simulink model "tokamak_integrated"  (R2026a)
settings: Solver=ode3  StopTime=30  FixedStep=1e-6  MaxStep=1e-5  RelTol=1e-5
model workspace (MAT data in the model file):
  load_L2 = 0.000636619772368
  load_R2 = 0.2
undefined symbols (not defined in the file): DiscIntNeverNeededParam
libraries: ee_lib x23, nesl_utility x19, fl_lib x11, gkc_lib x1
settings Model: ModifiedByFormat=GKC3-Simulink contributors  Creator=GKC3-Simulink contributors  LastModifiedBy=GKC3-Simulink contributors

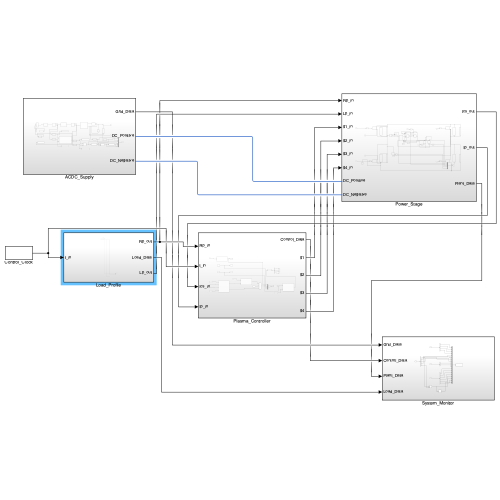
[thumbnail: Simulink's stored preview of the top-level diagram]
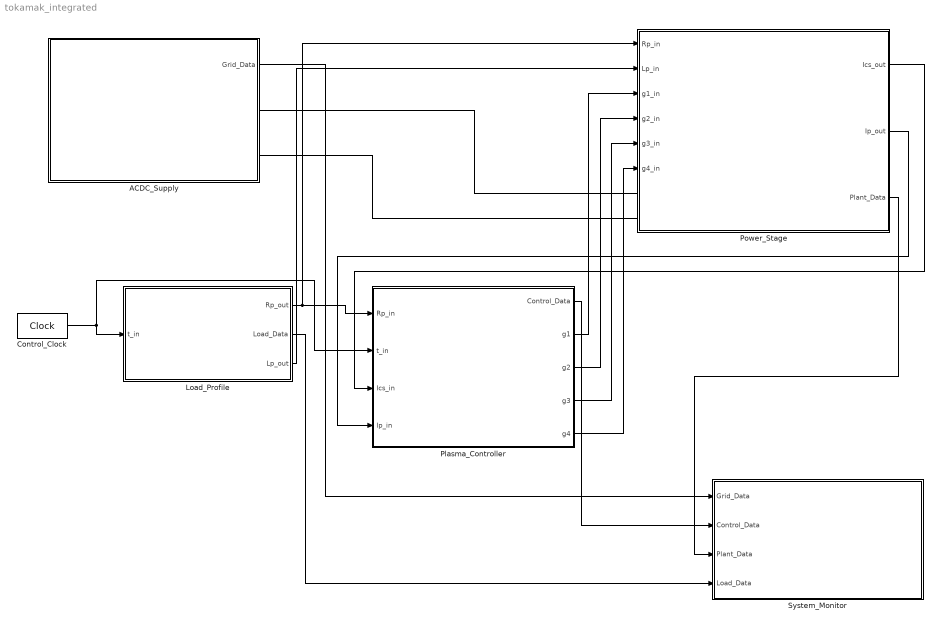
== system tokamak_integrated ==
  ACDC_Supply : Subsystem
  Control_Clock : DigitalClock  SampleTime=1e-5
  Load_Profile : Subsystem
  Plasma_Controller : Subsystem
  Power_Stage : Subsystem
  System_Monitor : Subsystem
  wires:
  Control_Clock/1 -> Load_Profile/1(t_in), Plasma_Controller/2(t_in)
  ACDC_Supply/1(Grid_Data) -> System_Monitor/1(Grid_Data)
  Plasma_Controller/1(Control_Data) -> System_Monitor/2(Control_Data)
  Plasma_Controller/2(g1) -> Power_Stage/3(g1_in)
  Plasma_Controller/3(g2) -> Power_Stage/4(g2_in)
  Plasma_Controller/4(g3) -> Power_Stage/5(g3_in)
  Plasma_Controller/5(g4) -> Power_Stage/6(g4_in)
  Power_Stage/1(Ics_out) -> Plasma_Controller/3(Ics_in)
  Power_Stage/2(Ip_out) -> Plasma_Controller/4(Ip_in)
  Power_Stage/3(Plant_Data) -> System_Monitor/3(Plant_Data)
  Load_Profile/1(Rp_out) -> Plasma_Controller/1(Rp_in), Power_Stage/1(Rp_in)
  Load_Profile/2(Load_Data) -> System_Monitor/4(Load_Data)
  Load_Profile/3(Lp_out) -> Power_Stage/2(Lp_in)
  connections:
  ACDC_Supply/RConn1 -- Power_Stage/LConn1
  ACDC_Supply/RConn2 -- Power_Stage/LConn2

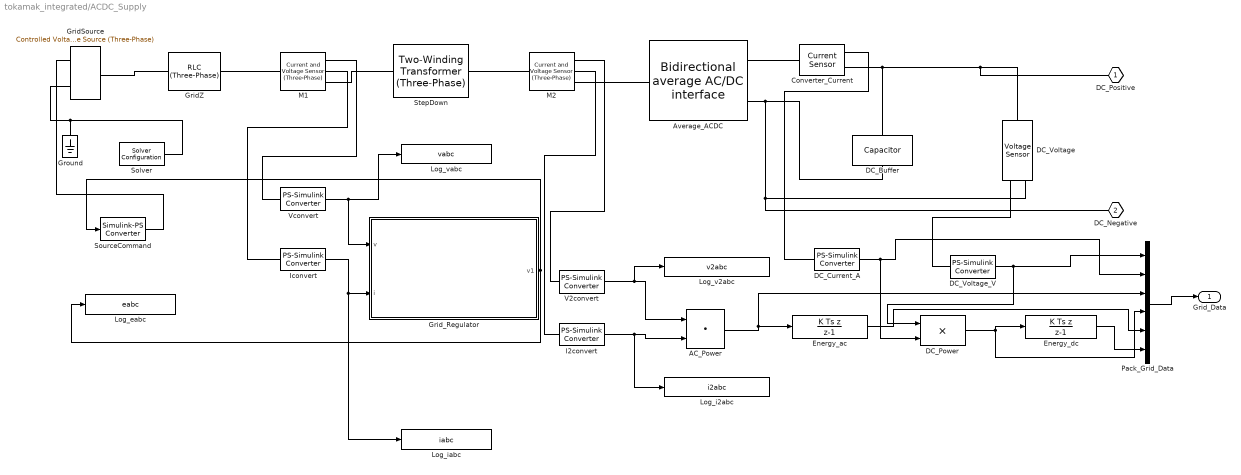
== system tokamak_integrated/ACDC_Supply ==
  AC_Power : DotProduct  OutDataTypeStr=Inherit: Inherit via internal rule
  Average_ACDC : gkc_lib/Bidirectional average AC//DC interface  voltage_ratio=2.2  frequency=50 Hz  phase=0 rad
  Converter_Current : fl_lib/Electrical/Electrical Sensors/Current Sensor
  DC_Buffer : ee_lib/Passive/Capacitor  cap_option=ee.enum.passive.capacitor.capOption.const  c=0.02 F  Cvec=[1e-05, 1e-06] F  Vvec=[0, 10] V  CV_table_symmetry=ee.enum.passive.capacitor.tableSymmetry.yes  f_vec=[1, 10] kHz  DFext_vec=[.8, 1.2]  enable_C_tol=ee.enum.toleranceApplication.none  averaging_period=0 s  C_tol=5  tol_distribution=ee.enum.toleranceDistribution.uniform  nSigma=4  r=0 Ohm  g=0 1/Ohm  enable_operating_limits=ee.enum.enable.no  operating_limit_action=ee.enum.passive.reportOpLim.warn  max_working_voltage_range=[-25, 25] V  power_rating=1 W  maxTemperature=85 degC  thermalEnable=false  thermalMass=1 J/K  i_specify=off  i_priority=None  i=0 A  i_nominal_specify=off  i_nominal_value=1  i_nominal_unit=A  v_specify=off  v_priority=None  v=0 V  v_nominal_specify=off  v_nominal_value=1  v_nominal_unit=V  vc_specify=on  vc_priority=High  vc=2200 V  vc_nominal_specify=off  vc_nominal_value=1  vc_nominal_unit=V  T_specify=off  T_priority=None  T=298.15 K  T_nominal_specify=off  T_nominal_value=1  T_nominal_unit=K
  DC_Current_A : nesl_utility/PS-Simulink Converter  PhysicalDomain=network_engine_domain  SubClassName=ps_output  LeftPortType=input  RightPortType=output  PseudoPeriodic=off  Frequencies=[]  VectorFormat=inherit  Unit=A  AffineConversion=off
  DC_Power : Product
  DC_Voltage : fl_lib/Electrical/Electrical Sensors/Voltage Sensor
  DC_Voltage_V : nesl_utility/PS-Simulink Converter  PhysicalDomain=network_engine_domain  SubClassName=ps_output  LeftPortType=input  RightPortType=output  PseudoPeriodic=off  Frequencies=[]  VectorFormat=inherit  Unit=V  AffineConversion=off
  Energy_ac : DiscreteIntegrator  IntegratorMethod=Integration: Backward Euler  SampleTime=1e-6  ICPrevOutput=DiscIntNeverNeededParam  ICPrevScaledInput=DiscIntNeverNeededParam
  Energy_dc : DiscreteIntegrator  IntegratorMethod=Integration: Backward Euler  SampleTime=1e-6  ICPrevOutput=DiscIntNeverNeededParam  ICPrevScaledInput=DiscIntNeverNeededParam
  GridSource : ee_lib/Sources/Controlled Voltage Source (Three-Phase)  Description=Implemented from the task-2 10 kV droop source guide.  input_option=ee.enum.inputType.instantaneous  FRated=50 Hz
  GridZ : ee_lib/Passive/RLC Assemblies/RLC (Three-Phase)  Description=Implemented from the task-2 10 kV droop source guide.  port_option=ee.enum.threePhasePort.composite  component_structure=ee.enum.rlc.structure.SeriesRL  R=0.1961161351 Ohm  L=0.0031212852 H  C=1e-6 F  R_parasitic=0 Ohm  G_parasitic=0 1/Ohm  IL_specify=off  IL_priority=High  IL=[0, 0, 0] A  IL_nominal_specify=off  IL_nominal_value=1  IL_nominal_unit=A  VC_specify=off  VC_priority=High  VC=[0, 0, 0] V  VC_nominal_specify=off  VC_nominal_value=1  VC_nominal_unit=V
  Grid_Regulator : Subsystem
  Ground : fl_lib/Electrical/Electrical Elements/Electrical Reference  Description=Implemented from the task-2 10 kV droop source guide.
  I2convert : nesl_utility/PS-Simulink Converter  Description=Implemented from the task-2 10 kV droop source guide.  PhysicalDomain=network_engine_domain  SubClassName=ps_output  LeftPortType=input  RightPortType=output  PseudoPeriodic=off  Frequencies=[]  VectorFormat=inherit  Unit=A  AffineConversion=off
  Iconvert : nesl_utility/PS-Simulink Converter  Description=Implemented from the task-2 10 kV droop source guide.  PhysicalDomain=network_engine_domain  SubClassName=ps_output  LeftPortType=input  RightPortType=output  PseudoPeriodic=off  Frequencies=[]  VectorFormat=inherit  Unit=A  AffineConversion=off
  Log_eabc : ToWorkspace  VariableName=eabc  SaveFormat=Timeseries  SampleTime=1e-4
      settings: Description=Implemented from the task-2 10 kV droop source guide.
  Log_i2abc : ToWorkspace  VariableName=i2abc  SaveFormat=Timeseries  SampleTime=1e-4
      settings: Description=Implemented from the task-2 10 kV droop source guide.
  Log_iabc : ToWorkspace  VariableName=iabc  SaveFormat=Timeseries  SampleTime=1e-4
      settings: Description=Implemented from the task-2 10 kV droop source guide.
  Log_v2abc : ToWorkspace  VariableName=v2abc  SaveFormat=Timeseries  SampleTime=1e-4
      settings: Description=Implemented from the task-2 10 kV droop source guide.
  Log_vabc : ToWorkspace  VariableName=vabc  SaveFormat=Timeseries  SampleTime=1e-4
      settings: Description=Implemented from the task-2 10 kV droop source guide.
  M1 : ee_lib/Sensors & Transducers/Current and Voltage Sensor (Three-Phase)  Description=10 kV bus measurement downstream of grid impedance; current positive toward load.  port_option=ee.enum.threePhasePort.composite  vMeasurementType=ee.enum.vmeasurement.lg  outputUnit=ee.enum.unit.si  SRated=100e6 A*V  VRated=24e3 V  I_specify=off  I_priority=None  I=[0, 0, 0] A  I_nominal_specify=off  I_nominal_value=1  I_nominal_unit=A  V_specify=off  V_priority=None  V=[0, 0, 0] V  V_nominal_specify=off  V_nominal_value=1  V_nominal_unit=V
  M2 : ee_lib/Sensors & Transducers/Current and Voltage Sensor (Three-Phase)  Description=Implemented from the task-2 10 kV droop source guide.  port_option=ee.enum.threePhasePort.composite  vMeasurementType=ee.enum.vmeasurement.lg  outputUnit=ee.enum.unit.si  SRated=100e6 A*V  VRated=24e3 V  I_specify=off  I_priority=None  I=[0, 0, 0] A  I_nominal_specify=off  I_nominal_value=1  I_nominal_unit=A  V_specify=off  V_priority=None  V=[0, 0, 0] V  V_nominal_specify=off  V_nominal_value=1  V_nominal_unit=V
  Pack_Grid_Data : Mux  Inputs=6
  Solver : nesl_utility/Solver Configuration  Description=Implemented from the task-2 10 kV droop source guide.  PhysicalDomain=network_engine_domain  SubClassName=solver  LeftPortType=input  RightPortType=generic  Tones=[]  Harmonics=[]  SimulateNoise=off  Profile=off  UseLocalSampling=off  EnableSwitchedLinearOptims=on  FrequencyDomain=off  UseCCode=off  RelTol=0.001  AbsTol=0.001  MinStep=1e-09  ToWorkspace=off  RevertToSquareIcSolve=off  NumHomotopyIterations=100  PhasorMode=off  PhasorModeNumHarmonics=1  ConsistencySolver=NEWTON_XTOL_AFTER_FTOL  CanonicalOrdering=CANONICAL  OptimizeIntermediates=OPTIMIZED  IndexReductionMethod=DerivativeReplacement  DoDC=off  ResidualTolerance=1e-09  ConsistencyTolSource=GLOBAL  ConsistencyAbsTol=0.001  ConsistencyRelTol=0.001  ConsistencyTolFactor=0.001  UseLocalSolver=on  LocalSolverChoice=NE_BACKWARD_EULER_ADVANCER  ResolveIndetEquations=on  FunctionEvalNumThread=1  LocalSolverSampleTime=1e-6  DoFixedCost=on  MaxNonlinIter=3  MaxModeIter=2  ComputeImpulses=off  ImpulseIterations=2  LinearAlgebra=Sparse  LinearAlgebraNumThread=0  EquationFormulation=NE_TIME_EF  DelaysMemoryBudget=1024  AutomaticFiltering=on  FilteringTimeConstant=0.001  PartitionStorageMethod=AS_NEEDED  PartitionMemoryBudget=1024  PartitionMethod=ROBUST  MultibodyUseLocalSolver=off  MultibodyLocalSolverChoice=ODE1  MultibodyLocalSolverSampleTime=0.001
  SourceCommand : nesl_utility/Simulink-PS Converter  Description=Implemented from the task-2 10 kV droop source guide.  PhysicalDomain=network_engine_domain  SubClassName=ps_input  LeftPortType=input  RightPortType=output  PseudoPeriodic=off  Frequencies=[]  NoiseDistribution=none  NoiseParameters=[]  Unit=V  AffineConversion=off  FilteringAndDerivatives=provide  SimscapeFilterOrder=1  InputFilterTimeConstant=0.001  UdotUserProvided=0
  StepDown : ee_lib/Passive/Transformers/Two-Winding Transformer (Three-Phase)  Description=Validation transformer: 10 kV/1000 V, 10 MVA, Yg/Yg, winding R 1e-6 pu each; no leakage/magnetization/saturation.  SRated=10e6 A*V  FRated=50 Hz  Winding1Connection=ee.enum.windingconnection.Yg  VRated1=10000 V  Winding2Connection=ee.enum.windingconnection.Yg  VRated2=1000 V  CoreType=ee.enum.coretype.threelimb  pu_Rw1=1e-6  pu_Rw2=1e-6  leakage_reactance_option=ee.enum.transformer_leakage.exclude  pu_Xl1=0.05  pu_Xl2=0.05  magnetizing_resistance_option=ee.enum.transformer_magnetizingResistance.exclude  pu_Rm=500  magnetizing_reactance_option=ee.enum.transformer_magnetizingReactance.exclude  saturation_option=ee.enum.transformer_saturation.exclude  pu_Xm=500  current_data=[0, .002, 1, 2]  magnetic_flux_data=[0, 1.2, 1.5, 1.51]  pu_X0=0.5  i1_specify=off  i1_priority=None  i1=[0, 0, 0] A  i1_nominal_specify=off  i1_nominal_value=1  i1_nominal_unit=A  i2_specify=off  i2_priority=None  i2=[0, 0, 0] A  i2_nominal_specify=off  i2_nominal_value=1  i2_nominal_unit=A  phi_specify=off  phi_priority=None  phi=[0, 0, 0]  phi_nominal_specify=off  phi_nominal_value=1  phi_nominal_unit=1
  V2convert : nesl_utility/PS-Simulink Converter  Description=Implemented from the task-2 10 kV droop source guide.  PhysicalDomain=network_engine_domain  SubClassName=ps_output  LeftPortType=input  RightPortType=output  PseudoPeriodic=off  Frequencies=[]  VectorFormat=inherit  Unit=V  AffineConversion=off
  Vconvert : nesl_utility/PS-Simulink Converter  Description=Implemented from the task-2 10 kV droop source guide.  PhysicalDomain=network_engine_domain  SubClassName=ps_output  LeftPortType=input  RightPortType=output  PseudoPeriodic=off  Frequencies=[]  VectorFormat=inherit  Unit=V  AffineConversion=off
  DC_Positive : PMIOPort  Side=Right
  DC_Negative : PMIOPort  Port=2  Side=Right
  Grid_Data : Outport
  wires:
  DC_Power/1 -> Pack_Grid_Data/4, Energy_dc/1
  Energy_dc/1 -> Pack_Grid_Data/6
  Pack_Grid_Data/1 -> Grid_Data/1
  DC_Current_A/1 -> Pack_Grid_Data/2, DC_Power/2
  AC_Power/1 -> Pack_Grid_Data/3, Energy_ac/1
  DC_Voltage_V/1 -> Pack_Grid_Data/1, DC_Power/1
  Energy_ac/1 -> Pack_Grid_Data/5
  Grid_Regulator/1(v1) -> SourceCommand/1, Log_eabc/1
  V2convert/1 -> Log_v2abc/1, AC_Power/1
  I2convert/1 -> Log_i2abc/1, AC_Power/2
  Iconvert/1 -> Log_iabc/1, Grid_Regulator/2(i)
  Vconvert/1 -> Log_vabc/1, Grid_Regulator/1(v)
  connections:
  DC_Voltage/RConn2 -- Average_ACDC/RConn2 -- DC_Buffer/RConn1 -- DC_Negative/RConn1
  Converter_Current/RConn2 -- DC_Positive/RConn1 -- DC_Voltage/LConn1 -- DC_Buffer/LConn1
  Solver/RConn1 -- Ground/LConn1 -- GridSource/LConn2
  M2/RConn2 -- I2convert/LConn1
  M1/RConn1 -- Vconvert/LConn1
  GridZ/RConn1 -- M1/LConn1
  M1/RConn3 -- StepDown/LConn1
  GridSource/RConn1 -- GridZ/LConn1
  StepDown/RConn1 -- M2/LConn1
  DC_Voltage/RConn1 -- DC_Voltage_V/LConn1
  M2/RConn1 -- V2convert/LConn1
  M1/RConn2 -- Iconvert/LConn1
  SourceCommand/RConn1 -- GridSource/LConn1
  Average_ACDC/RConn1 -- Converter_Current/LConn1
  Converter_Current/RConn1 -- DC_Current_A/LConn1
  M2/RConn3 -- Average_ACDC/LConn1

== system tokamak_integrated/Load_Profile ==
  t_in : Inport
  Lp_schedule : Lookup_n-D  NumberOfTableDimensions=1  BreakpointsForDimension1=[0 0.6 1.6 30]  Table=[150e-6 150e-6 100e-6 100e-6]  ExtrapMethod=Clip  InternalRulePriority=Speed  RndMeth=Simplest
  Pack_Load_Data : Mux  Inputs=2
  Rp_schedule : Lookup_n-D  NumberOfTableDimensions=1  BreakpointsForDimension1=[0 0.6 1.6 11.6 12.1 12.3 30]  Table=[0.015 0.015 0.01 0.01 0.01 100 100]  ExtrapMethod=Clip  InternalRulePriority=Speed  RndMeth=Simplest
  Rp_out : Outport
  Load_Data : Outport  Port=2
  Lp_out : Outport  Port=3
  wires:
  Rp_schedule/1 -> Pack_Load_Data/1, Rp_out/1
  Pack_Load_Data/1 -> Load_Data/1
  Lp_schedule/1 -> Lp_out/1, Pack_Load_Data/2
  t_in/1 -> Rp_schedule/1, Lp_schedule/1

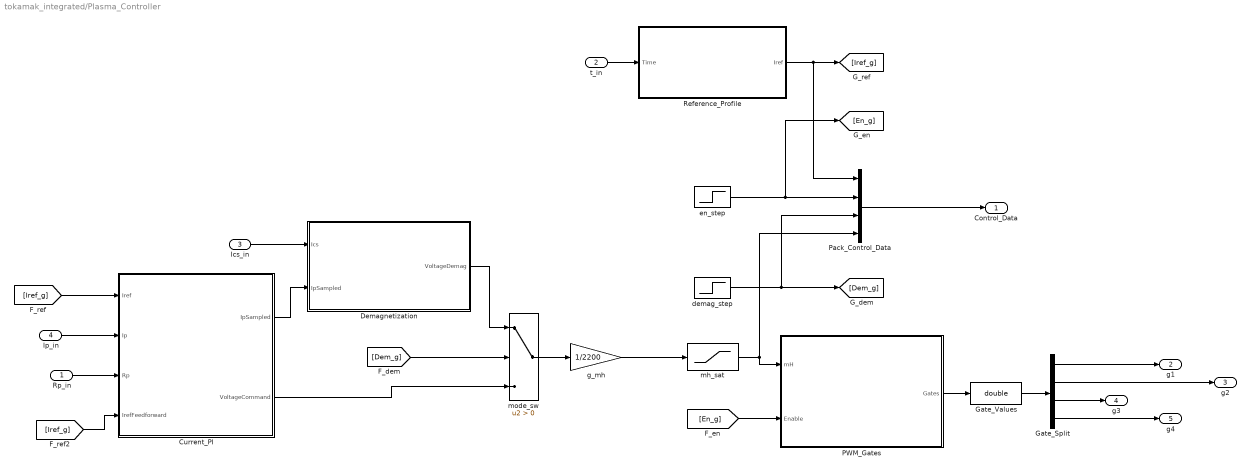
== system tokamak_integrated/Plasma_Controller ==
  Rp_in : Inport
  t_in : Inport  Port=2
  Ics_in : Inport  Port=3
  Ip_in : Inport  Port=4
  Current_PI : Subsystem
  Demagnetization : Subsystem
  Gate_Split : Demux
  Gate_Values : DataTypeConversion  OutDataTypeStr=double  SaturateOnIntegerOverflow=off  RndMeth=Floor
  PWM_Gates : Subsystem
  Pack_Control_Data : Mux
  Reference_Profile : Subsystem
  demag_step : Step  Time=12.3  SampleTime=0
  en_step : Step  Time=0.6  SampleTime=0
  g_mh : Gain  Gain=1/2200
  mh_sat : Saturate  UpperLimit=0.95  LowerLimit=-0.95
  mode_sw : Switch  Criteria=u2 > Threshold  SaturateOnIntegerOverflow=off  InputSameDT=off
  Control_Data : Outport
  g1 : Outport  Port=2
  g2 : Outport  Port=3
  g3 : Outport  Port=4
  g4 : Outport  Port=5
  wires:
  g_mh/1 -> mh_sat/1
  t_in/1 -> Reference_Profile/1(Time)
  [Iref_g] -> Current_PI/1(Iref)
  Ip_in/1 -> Current_PI/2(Ip)
  Rp_in/1 -> Current_PI/3(Rp)
  [Iref_g] -> Current_PI/4(IrefFeedforward)
  Current_PI/2(VoltageCommand) -> mode_sw/3
  Ics_in/1 -> Demagnetization/1(Ics)
  Current_PI/1(IpSampled) -> Demagnetization/2(IpSampled)
  Demagnetization/1(VoltageDemag) -> mode_sw/1
  [En_g] -> PWM_Gates/2(Enable)
  [Dem_g] -> mode_sw/2
  mode_sw/1 -> g_mh/1
  Pack_Control_Data/1 -> Control_Data/1
  Gate_Split/3 -> g3/1
  Gate_Split/1 -> g1/1
  PWM_Gates/1(Gates) -> Gate_Values/1
  Reference_Profile/1(Iref) -> [Iref_g], Pack_Control_Data/1
  mh_sat/1 -> PWM_Gates/1(mH), Pack_Control_Data/4
  Gate_Split/2 -> g2/1
  Gate_Split/4 -> g4/1
  Gate_Values/1 -> Gate_Split/1
  en_step/1 -> [En_g], Pack_Control_Data/2
  demag_step/1 -> [Dem_g], Pack_Control_Data/3

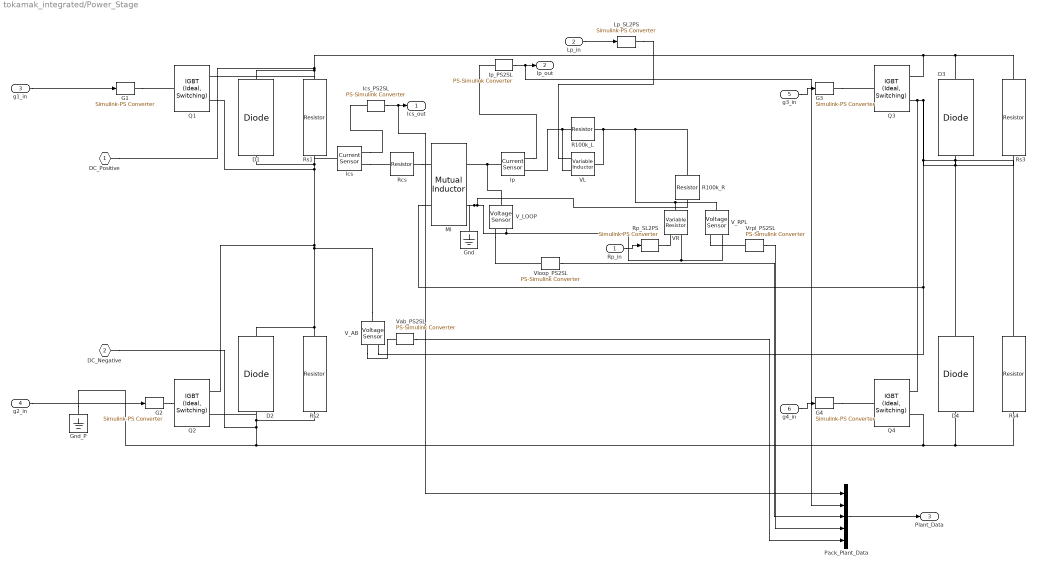
== system tokamak_integrated/Power_Stage ==
  Rp_in : Inport
  Lp_in : Inport  Port=2
  g1_in : Inport  Port=3
  g2_in : Inport  Port=4
  g3_in : Inport  Port=5
  g4_in : Inport  Port=6
  D{1..4} (4 alike) : ee_lib/Semiconductors & Converters/Diode  ModelType=ee.enum.diode.modelType.pwl  TableType=ee.enum.diode.tableType.IfMat  IfMat=[.07, .12, .19, 1.75, 4.24, 7.32, 11.2; .16, .3, .72, 2.14, 5.02, 8.35, 13.12] A  VfMat=[.9, 1.15, 1.25, 1.5, 1.75, 2.17, 2.6, 2.85; .58, .68, .75, 1.1, 1.38, 1.77, 2.27, 2.7] V  TjVec=[25, 125] degC  VfVec=[.5, .7, .9, 1.3, 1.7, 2.1, 2.5] V  IfVec=[.1, .2, .5, 1, 2, 4, 7, 10] A  IrMat=[1e-06, 2e-06, 5e-06, 1e-05, 2.5e-05, 5e-05, .0001; 2e-06, 5e-06, 1e-05, 4e-05, 8e-05, .0002, .0005] A  VrMat=[10, 100, 200, 250, 300, 325, 350; 10, 70, 160, 220, 270, 300, 320] V  VrVec=[10, 20, 40, 50, 70, 80, 100] V  IrVec=[1e-06, 2e-06, 5e-06, 1e-05, 2e-05, 5e-05, .0001] A  Vf=2 V  Ron=20e-6 Ohm  Goff=1e-8 S  prmExp=ee.enum.diode.expParam.useTwo  I12=[.0137, .545] A  V12=[.6, .7] V  RS=0 Ohm  Tmeas=298.15 K  IS=1e-12 A  ec=1  I1=0.0137 A  V1=0.6 V  N_series=1  N_parallel=1  ZenerEnable=false  Rz=0.3 Ohm  BV=30 V  C_param=ee.enum.diode.capParam.fixed  CJ=0 pF  CJ0=5 pF  Vvec=[.1, 10, 100] V  Cvec=[3.5, 1, .4] pF  VJ=1 V  Mgrad=0.5  FC=0.5  Q_param=ee.enum.diode.recoveryParam.off  iRM=-7.15 A  iF=4 A  didt=-750 A/us  trr_factor=3  trr=115 ns  Qrr=150 nA*s  Vr=-600 V  Ls=150 nH  Erec=0.03 J  TT=50 ns  tau=100 ns  T_param=ee.enum.diode.temperatureParam.off  Tdevice=298.15 K  I1_T2=0.245 A  V1_T2=0.5 V  IS_T2=1.25e-7 A  Tmeas2=125 degC  XTI_param=ee.enum.diode.xtiParam.pn  XTI=3  EG_param=ee.enum.diode.egapParam.material_si  EG=1.11 eV  dBVdT=0 V/K  enable_fault_input=simscape.enum.onoff.off  i_specify=off  i_priority=None  i=0 A  i_nominal_specify=off  i_nominal_value=1  i_nominal_unit=A  v_specify=off  v_priority=None  v=0 V  v_nominal_specify=off  v_nominal_value=1  v_nominal_unit=V  v_capacitor_specify=off  v_capacitor_priority=None  v_capacitor=0 V  v_capacitor_nominal_specify=off  v_capacitor_nominal_value=1  v_capacitor_nominal_unit=V  Qj_specify=off  Qj_priority=High  Qj=0 C  Qj_nominal_specify=off  Qj_nominal_value=1  Qj_nominal_unit=C  i_diode_specify=off  i_diode_priority=None  i_diode=0 A  i_diode_nominal_specify=off  i_diode_nominal_value=1  i_diode_nominal_unit=A  v_diode_specify=off  v_diode_priority=None  v_diode=0 V  v_diode_nominal_specify=off  v_diode_nominal_value=1  v_diode_nominal_unit=V  i_capacitor_specify=off  i_capacitor_priority=None  i_capacitor=0 A  i_capacitor_nominal_specify=off  i_capacitor_nominal_value=1  i_capacitor_nominal_unit=A  fidelity_level=ee.enum.diode.fidelity.includeChargeDyn  rec_loss_model=ee.enum.diode.reverseRecoveryModelTabulateUpTo3D.fixed  ErecVal=0 J  scaleWithIandV=true  ErecMat=zeros(2, 3) J  ErecMat3D=zeros(2, 3, 2) J  TjrecVec=[298.15, 398.15] K  IfrecVec=[.1, 1, 10] A  IrecVal=10 A  VrecVal=10 V  VrecVec=[0, 100] V  tFilter=1 / 1000 / 100 s  thermal_network_parameterization=ee.enum.thermalNetworkTopology.junctionCase  Rth=[0, 10] K/W  Rth_Cauer=[1, 3, 10] K/W  Rth_Foster=[.08, .14, .22, .16] K/W  thermal_mass_parameterization=ee.enum.thermalNetwork.timeconstant  thermal_mass=[0, 1] J/K  thermal_mass_Cauer=[.1, .3, 1] J/K  thermal_mass_Foster=[.001, .005, .05, .5] J/K  thermal_time_constant=[0, 10] s  thermal_time_constant_Cauer=[1, 3, 10] s  thermal_time_constant_Foster=[7e-05, .0007, .01, .08] s  thermal_mass_initial_temperatures=[25, 25] degC  thermal_mass_initial_temperatures_Cauer=[25, 25, 25] degC  junction_thermal_mass=0.01 J/K  Tvec_initial_Foster=[25, 25, 25, 25] degC  no_thermal_network=0  junction_temperature_specify=off  junction_temperature_priority=None  junction_temperature=25 degC  junction_temperature_nominal_specify=off  junction_temperature_nominal_value=1  junction_temperature_nominal_unit=degC
  G{1..4} (4 alike) : nesl_utility/Simulink-PS Converter  PhysicalDomain=network_engine_domain  SubClassName=ps_input  LeftPortType=input  RightPortType=output  PseudoPeriodic=off  Frequencies=[]  NoiseDistribution=none  NoiseParameters=[]  Unit=V  AffineConversion=off  FilteringAndDerivatives=zero  SimscapeFilterOrder=1  InputFilterTimeConstant=0.001  UdotUserProvided=0
  Gnd : fl_lib/Electrical/Electrical Elements/Electrical Reference
  Gnd_P : fl_lib/Electrical/Electrical Elements/Electrical Reference
  Ics : fl_lib/Electrical/Electrical Sensors/Current Sensor
  Ics_PS2SL : nesl_utility/PS-Simulink Converter  PhysicalDomain=network_engine_domain  SubClassName=ps_output  LeftPortType=input  RightPortType=output  PseudoPeriodic=off  Frequencies=[]  VectorFormat=inherit  Unit=A  AffineConversion=off
  Ip : fl_lib/Electrical/Electrical Sensors/Current Sensor
  Ip_PS2SL : nesl_utility/PS-Simulink Converter  PhysicalDomain=network_engine_domain  SubClassName=ps_output  LeftPortType=input  RightPortType=output  PseudoPeriodic=off  Frequencies=[]  VectorFormat=inherit  Unit=A  AffineConversion=off
  Lp_SL2PS : nesl_utility/Simulink-PS Converter  PhysicalDomain=network_engine_domain  SubClassName=ps_input  LeftPortType=input  RightPortType=output  PseudoPeriodic=off  Frequencies=[]  NoiseDistribution=none  NoiseParameters=[]  Unit=H  AffineConversion=off  FilteringAndDerivatives=provide  SimscapeFilterOrder=1  InputFilterTimeConstant=0.001  UdotUserProvided=0
  MI : ee_lib/Passive/Transformers/Mutual Inductor  L1=1 H  L2=1 H  k=0.99999  L_tol=20  enable_L1_tol=ee.enum.toleranceApplication.none  L1_tol_distribution=ee.enum.toleranceDistribution.uniform  L1_nSigma=4  enable_L2_tol=ee.enum.toleranceApplication.none  L2_tol_distribution=ee.enum.toleranceDistribution.uniform  L2_nSigma=4  r=[1e-9, 1e-9] Ohm  g=[1e-9, 1e-9] 1/Ohm  enable_operating_limits=ee.enum.enable.no  operating_limit_action=ee.enum.passive.reportOpLim.warn  max_working_current=1 A  power_rating=1 W  iL1_specify=off  iL1_priority=High  iL1=0 A  iL1_nominal_specify=off  iL1_nominal_value=1  iL1_nominal_unit=A  iL2_specify=off  iL2_priority=High  iL2=0 A  iL2_nominal_specify=off  iL2_nominal_value=1  iL2_nominal_unit=A
  Pack_Plant_Data : Mux  Inputs=5
  Q{1..4} (4 alike) : ee_lib/Semiconductors & Converters/IGBT (Ideal, Switching)  port_option=ee.enum.controlport.ps  Vf=2 V  Ron=20e-6 Ohm  Goff=1e-8 1/Ohm  Vth=0.5 V  diode_param=ee.enum.semiconductors.protectionDiode.external  diode_Vf=0.8 V  diode_Ron=0.001 Ohm  diode_Goff=1e-5 1/Ohm  diode_C=50e-9 F  diode_iRM=-235 A  diode_iF=300 A  diode_idot=-50 A/us  diode_trr_param=ee.enum.converters.diodeReverseParam.trr_factor  diode_trr_factor=3  diode_trr=15 us  diode_Qrr=1500 s*uA  ice_specify=off  ice_priority=None  ice=0 A  ice_nominal_specify=off  ice_nominal_value=1  ice_nominal_unit=A  vce_specify=off  vce_priority=None  vce=0 V  vce_nominal_specify=off  vce_nominal_value=1  vce_nominal_unit=V  vge_specify=off  vge_priority=None  vge=0 V  vge_nominal_specify=off  vge_nominal_value=1  vge_nominal_unit=V  thermal_loss_option=ee.enum.converters.thermalLossOption.constantvalues  Von_data=[0, .1, .6, .8, 1, 1.3, 1.6, 2, 2.4; 0, .1, .7, 1, 1.2, 1.5, 1.9, 2.4, 2.8] V  Tj=[298.15, 398.15] K  Iout_data=[0, .1, 1, 5, 10, 20, 40, 70, 100] A  tabulateWithVce=false  Eon_data=[0, .0024, .024, .12, .2, .48, 1.04, 2.16, 3.24; 0, .003, .03, .15, .25, .6, 1.3, 2.7, 4.05] * 1e-3 J  Eoff_data=[0, .0007, .0066, .033, .066, .17, .33, .83, 1.5; 0, .001, .01, .05, .1, .25, .5, 1.2, 2.2] * 1e-3 J  Eon_data_3D=[zeros(2, 9, 3)] J  Eoff_data_3D=[zeros(2, 9, 3)] J  Tj_loss=[298.15, 398.15] K  Iout_data_loss=[0, .1, 1, 5, 10, 20, 40, 70, 100] A  Vce_loss=[0, 150, 300] V  Eon_scalar=22.86e-3 J  Eoff_scalar=17.14e-3 J  Voff=300 V  Iout_scalar=600 A  useCurrentFromPreviousCycle=false  useVoltageFromPreviousCycle=false  diodeModelType=ee.enum.converters.diodeModelType.pwl  diodeTableType=ee.enum.diode.tableType.IfMat  diode_ReverseIVType=ee.enum.diode.diodeReverseIV.constant  diode_IfMat=[.07, .12, .19, 1.75, 4.24, 7.32, 11.2; .16, .3, .72, 2.14, 4.02, 6.35, 9.12] A  diode_VfMat=[.9, 1.15, 1.25, 1.5, 1.75, 2.17, 2.6, 2.85; .58, .68, .75, 1.1, 1.38, 1.77, 2.27, 2.7] V  diode_TjVec=[25, 125] degC  diode_VfVec=[.5, .7, .9, 1.3, 1.7, 2.1, 2.5] V  diode_IfVec=[.1, .2, .5, 1, 2, 4, 7, 10] A  diode_IrMat=[1e-06, 2e-06, 5e-06, 1e-05, 2.5e-05, 5e-05, .0001; 2e-06, 5e-06, 1e-05, 4e-05, 8e-05, .0002, .0005] A  diode_VrMat=[10, 100, 200, 250, 300, 325, 350; 10, 70, 160, 220, 270, 300, 320] V  diode_VrVec=[10, 20, 40, 50, 70, 80, 100] V  diode_IrVec=[1e-06, 2e-06, 5e-06, 1e-05, 2e-05, 5e-05, .0001] A  diode_Vr=-600 V  diode_Ls=150 nH  diode_Erec=0.03 J  diode_rec_loss_model=ee.enum.diode.reverseRecoveryModelTabulateUpTo3D.fixed  diode_ErecVal=0 J  diode_scaleWithIandV=true  diode_ErecMat=zeros(2, 3) J  diodeErecMat3D=zeros(2, 3, 2) J  diode_TjrecVec=[298.15, 398.15] K  diode_IfrecVec=[.1, 1, 10] A  diodeVrecVec=[0, 100] V  diode_IrecVal=10 A  diode_VrecVal=10 V  diode_tFilter=1 / 1000 / 100 s  separateThermalPortForDiode=false  thermal_network_parameterization=ee.enum.thermalNetworkTopology.external  Rth=[.08, .5] K/W  Rth_Cauer=[.08, .1, .5] K/W  Rth_Foster=[.08, .14, .22, .16] K/W  thermal_mass_parameterization=ee.enum.thermalNetwork.timeconstant  thermal_mass=[.01, .5] J/K  thermal_mass_Cauer=[.01, .1, .5] J/K  thermal_mass_Foster=[.001, .005, .05, .5] J/K  thermal_time_constant=[.001, .2] s  thermal_time_constant_Cauer=[.001, .1, .2] s  thermal_time_constant_Foster=[7e-05, .0007, .01, .08] s  thermal_mass_initial_temperatures=[25, 25] degC  thermal_mass_initial_temperatures_Cauer=[25, 25, 25] degC  junction_thermal_mass=0.01 J/K  Tvec_initial_Foster=[25, 25, 25, 25] degC  RthDiode=[.03, .2] K/W  RthCauerDiode=[.03, .1, .2] K/W  RthFosterDiode=[.03, .2] K/W  thermalMassDiode=[3, 25] J/K  thermalMassCauerDiode=[3, 10, 25] J/K  thermalMassFosterDiode=[33, 50] J/K  thermalTauDiode=[.1, 5] s  thermalTauCauerDiode=[.1, 1, 5] s  thermalTauFosterDiode=[1, 10] s  thermalMassInitTempDiode=[25, 25] degC  thermalMassInitTempCauerDiode=[25, 25, 25] degC  junctionthermalMassDiode=0.1 J/K  TVecInitialFosterDiode=[25, 25, 25, 25] degC  no_thermal_network=ee.enum.enable.no  IGBT_junction_temperature_specify=off  IGBT_junction_temperature_priority=None  IGBT_junction_temperature=25 degC  IGBT_junction_temperature_nominal_specify=off  IGBT_junction_temperature_nominal_value=1  IGBT_junction_temperature_nominal_unit=degC  diode_junction_temperature_specify=off  diode_junction_temperature_priority=None  diode_junction_temperature=25 degC  diode_junction_temperature_nominal_specify=off  diode_junction_temperature_nominal_value=1  diode_junction_temperature_nominal_unit=degC  Qj_specify=off  Qj_priority=None  Qj=0 W  Qj_nominal_specify=off  Qj_nominal_value=1  Qj_nominal_unit=W  accumulatedSwitchingLosses_specify=off  accumulatedSwitchingLosses_priority=None  accumulatedSwitchingLosses=0 J
  R100k_L : ee_lib/Passive/Resistor  R=1e5 Ohm  enable_R_tol=ee.enum.toleranceApplication.none  R_tol=5  tol_distribution=ee.enum.toleranceDistribution.uniform  nSigma=4  enable_operating_limits=ee.enum.enable.no  operating_limit_action=ee.enum.passive.reportOpLim.warn  power_rating=1 W  max_working_voltage=100 V  noise_mode=ee.enum.sources.noise.Disabled  Tdevice=25 degC  sample_time=1e-3 s  repeatability=ee.enum.ic.repeatability.notRepeatable  user_seed=0  auto_seed=817904655  power_derating_T1=70 degC  power_derating_T2=155 degC  operating_temperature_range_vec=[-50, 150] degC  alpha=3.93e-3 1/K  Tmeas=25 degC  thermal_mass=100 J/K  temperature_specify=off  temperature_priority=High  temperature=298.15 K  temperature_nominal_specify=off  temperature_nominal_value=1  temperature_nominal_unit=K
  R100k_R : ee_lib/Passive/Resistor  R=1e5 Ohm  enable_R_tol=ee.enum.toleranceApplication.none  R_tol=5  tol_distribution=ee.enum.toleranceDistribution.uniform  nSigma=4  enable_operating_limits=ee.enum.enable.no  operating_limit_action=ee.enum.passive.reportOpLim.warn  power_rating=1 W  max_working_voltage=100 V  noise_mode=ee.enum.sources.noise.Disabled  Tdevice=25 degC  sample_time=1e-3 s  repeatability=ee.enum.ic.repeatability.notRepeatable  user_seed=0  auto_seed=1584484500  power_derating_T1=70 degC  power_derating_T2=155 degC  operating_temperature_range_vec=[-50, 150] degC  alpha=3.93e-3 1/K  Tmeas=25 degC  thermal_mass=100 J/K  temperature_specify=off  temperature_priority=High  temperature=298.15 K  temperature_nominal_specify=off  temperature_nominal_value=1  temperature_nominal_unit=K
  Rcs : ee_lib/Passive/Resistor  R=20e-6 Ohm  enable_R_tol=ee.enum.toleranceApplication.none  R_tol=5  tol_distribution=ee.enum.toleranceDistribution.uniform  nSigma=4  enable_operating_limits=ee.enum.enable.no  operating_limit_action=ee.enum.passive.reportOpLim.warn  power_rating=1 W  max_working_voltage=100 V  noise_mode=ee.enum.sources.noise.Disabled  Tdevice=25 degC  sample_time=1e-3 s  repeatability=ee.enum.ic.repeatability.notRepeatable  user_seed=0  auto_seed=1978802833  power_derating_T1=70 degC  power_derating_T2=155 degC  operating_temperature_range_vec=[-50, 150] degC  alpha=3.93e-3 1/K  Tmeas=25 degC  thermal_mass=100 J/K  temperature_specify=off  temperature_priority=High  temperature=298.15 K  temperature_nominal_specify=off  temperature_nominal_value=1  temperature_nominal_unit=K
  Rp_SL2PS : nesl_utility/Simulink-PS Converter  PhysicalDomain=network_engine_domain  SubClassName=ps_input  LeftPortType=input  RightPortType=output  PseudoPeriodic=off  Frequencies=[]  NoiseDistribution=none  NoiseParameters=[]  Unit=Ohm  AffineConversion=off  FilteringAndDerivatives=provide  SimscapeFilterOrder=1  InputFilterTimeConstant=0.001  UdotUserProvided=0
  Rs1 : ee_lib/Passive/Resistor  R=1e7 Ohm  enable_R_tol=ee.enum.toleranceApplication.none  R_tol=5  tol_distribution=ee.enum.toleranceDistribution.uniform  nSigma=4  enable_operating_limits=ee.enum.enable.no  operating_limit_action=ee.enum.passive.reportOpLim.warn  power_rating=1 W  max_working_voltage=100 V  noise_mode=ee.enum.sources.noise.Disabled  Tdevice=25 degC  sample_time=1e-3 s  repeatability=ee.enum.ic.repeatability.notRepeatable  user_seed=0  auto_seed=4216102895  power_derating_T1=70 degC  power_derating_T2=155 degC  operating_temperature_range_vec=[-50, 150] degC  alpha=3.93e-3 1/K  Tmeas=25 degC  thermal_mass=100 J/K  temperature_specify=off  temperature_priority=High  temperature=298.15 K  temperature_nominal_specify=off  temperature_nominal_value=1  temperature_nominal_unit=K
  Rs2 : ee_lib/Passive/Resistor  R=1e7 Ohm  enable_R_tol=ee.enum.toleranceApplication.none  R_tol=5  tol_distribution=ee.enum.toleranceDistribution.uniform  nSigma=4  enable_operating_limits=ee.enum.enable.no  operating_limit_action=ee.enum.passive.reportOpLim.warn  power_rating=1 W  max_working_voltage=100 V  noise_mode=ee.enum.sources.noise.Disabled  Tdevice=25 degC  sample_time=1e-3 s  repeatability=ee.enum.ic.repeatability.notRepeatable  user_seed=0  auto_seed=671754155  power_derating_T1=70 degC  power_derating_T2=155 degC  operating_temperature_range_vec=[-50, 150] degC  alpha=3.93e-3 1/K  Tmeas=25 degC  thermal_mass=100 J/K  temperature_specify=off  temperature_priority=High  temperature=298.15 K  temperature_nominal_specify=off  temperature_nominal_value=1  temperature_nominal_unit=K
  Rs3 : ee_lib/Passive/Resistor  R=1e7 Ohm  enable_R_tol=ee.enum.toleranceApplication.none  R_tol=5  tol_distribution=ee.enum.toleranceDistribution.uniform  nSigma=4  enable_operating_limits=ee.enum.enable.no  operating_limit_action=ee.enum.passive.reportOpLim.warn  power_rating=1 W  max_working_voltage=100 V  noise_mode=ee.enum.sources.noise.Disabled  Tdevice=25 degC  sample_time=1e-3 s  repeatability=ee.enum.ic.repeatability.notRepeatable  user_seed=0  auto_seed=3674442472  power_derating_T1=70 degC  power_derating_T2=155 degC  operating_temperature_range_vec=[-50, 150] degC  alpha=3.93e-3 1/K  Tmeas=25 degC  thermal_mass=100 J/K  temperature_specify=off  temperature_priority=High  temperature=298.15 K  temperature_nominal_specify=off  temperature_nominal_value=1  temperature_nominal_unit=K
  Rs4 : ee_lib/Passive/Resistor  R=1e7 Ohm  enable_R_tol=ee.enum.toleranceApplication.none  R_tol=5  tol_distribution=ee.enum.toleranceDistribution.uniform  nSigma=4  enable_operating_limits=ee.enum.enable.no  operating_limit_action=ee.enum.passive.reportOpLim.warn  power_rating=1 W  max_working_voltage=100 V  noise_mode=ee.enum.sources.noise.Disabled  Tdevice=25 degC  sample_time=1e-3 s  repeatability=ee.enum.ic.repeatability.notRepeatable  user_seed=0  auto_seed=2769242599  power_derating_T1=70 degC  power_derating_T2=155 degC  operating_temperature_range_vec=[-50, 150] degC  alpha=3.93e-3 1/K  Tmeas=25 degC  thermal_mass=100 J/K  temperature_specify=off  temperature_priority=High  temperature=298.15 K  temperature_nominal_specify=off  temperature_nominal_value=1  temperature_nominal_unit=K
  VL : ee_lib/Passive/Variable Inductor  prm=1  Lmin=1e-6 H  g=1e-9 1/Ohm  i0=0 A  phi0=0 Wb
  VR : fl_lib/Electrical/Electrical Elements/Variable Resistor  Rmin=1e-5 Ohm  thermalEnable=false  thermal_mass=1 J/K  i_specify=off  i_priority=None  i=0 A  i_nominal_specify=off  i_nominal_value=1  i_nominal_unit=A  v_specify=off  v_priority=None  v=0 V  v_nominal_specify=off  v_nominal_value=1  v_nominal_unit=V  T_specify=off  T_priority=None  T=300 K  T_nominal_specify=off  T_nominal_value=1  T_nominal_unit=K
  V_AB : fl_lib/Electrical/Electrical Sensors/Voltage Sensor
  V_LOOP : fl_lib/Electrical/Electrical Sensors/Voltage Sensor
  V_RPL : fl_lib/Electrical/Electrical Sensors/Voltage Sensor
  Vab_PS2SL : nesl_utility/PS-Simulink Converter  PhysicalDomain=network_engine_domain  SubClassName=ps_output  LeftPortType=input  RightPortType=output  PseudoPeriodic=off  Frequencies=[]  VectorFormat=inherit  Unit=V  AffineConversion=off
  Vloop_PS2SL : nesl_utility/PS-Simulink Converter  PhysicalDomain=network_engine_domain  SubClassName=ps_output  LeftPortType=input  RightPortType=output  PseudoPeriodic=off  Frequencies=[]  VectorFormat=inherit  Unit=V  AffineConversion=off
  Vrpl_PS2SL : nesl_utility/PS-Simulink Converter  PhysicalDomain=network_engine_domain  SubClassName=ps_output  LeftPortType=input  RightPortType=output  PseudoPeriodic=off  Frequencies=[]  VectorFormat=inherit  Unit=V  AffineConversion=off
  DC_Positive : PMIOPort  Side=Left
  DC_Negative : PMIOPort  Port=2  Side=Left
  Ics_out : Outport
  Ip_out : Outport  Port=2
  Plant_Data : Outport  Port=3
  wires:
  Vrpl_PS2SL/1 -> Pack_Plant_Data/4
  Pack_Plant_Data/1 -> Plant_Data/1
  Ics_PS2SL/1 -> Ics_out/1, Pack_Plant_Data/1
  Vloop_PS2SL/1 -> Pack_Plant_Data/3
  Vab_PS2SL/1 -> Pack_Plant_Data/5
  Ip_PS2SL/1 -> Ip_out/1, Pack_Plant_Data/2
  Rp_in/1 -> Rp_SL2PS/1
  Lp_in/1 -> Lp_SL2PS/1
  g4_in/1 -> G4/1
  g3_in/1 -> G3/1
  g2_in/1 -> G2/1
  g1_in/1 -> G1/1
  connections:
  G1/RConn1 -- Q1/LConn1
  G3/RConn1 -- Q3/LConn1
  Rcs/RConn1 -- MI/LConn1
  VR/LConn2 -- Gnd/LConn1 -- MI/RConn2 -- R100k_R/LConn1 -- V_LOOP/RConn2 -- V_RPL/RConn2
  MI/RConn1 -- Ip/LConn1 -- V_LOOP/LConn1
  MI/LConn2 -- D3/LConn1 -- Rs3/LConn1 -- Rs4/RConn1 -- D4/RConn1 -- Q4/RConn1 -- Q3/RConn2 -- V_AB/RConn2
  V_AB/LConn1 -- Rs2/RConn1 -- D2/RConn1 -- Rs1/LConn1 -- D1/LConn1 -- Ics/LConn1 -- Q1/RConn2 -- Q2/RConn1
  Gnd_P/LConn1 -- Rs4/LConn1 -- D4/LConn1 -- Q4/RConn2 -- Q2/RConn2 -- D2/LConn1 -- Rs2/LConn1 -- DC_Negative/RConn1
  Q3/RConn1 -- D1/RConn1 -- Q1/RConn1 -- Rs1/RConn1 -- DC_Positive/RConn1 -- Rs3/RConn1 -- D3/RConn1
  VL/LConn2 -- R100k_L/LConn1 -- Ip/RConn2
  VR/RConn1 -- VL/RConn1 -- R100k_L/RConn1 -- R100k_R/RConn1 -- V_RPL/LConn1
  V_AB/RConn1 -- Vab_PS2SL/LConn1
  V_RPL/RConn1 -- Vrpl_PS2SL/LConn1
  V_LOOP/RConn1 -- Vloop_PS2SL/LConn1
  Ip/RConn1 -- Ip_PS2SL/LConn1
  Ics/RConn1 -- Ics_PS2SL/LConn1
  Rp_SL2PS/RConn1 -- VR/LConn1
  Lp_SL2PS/RConn1 -- VL/LConn1
  Ics/RConn2 -- Rcs/LConn1
  G4/RConn1 -- Q4/LConn1
  G2/RConn1 -- Q2/LConn1

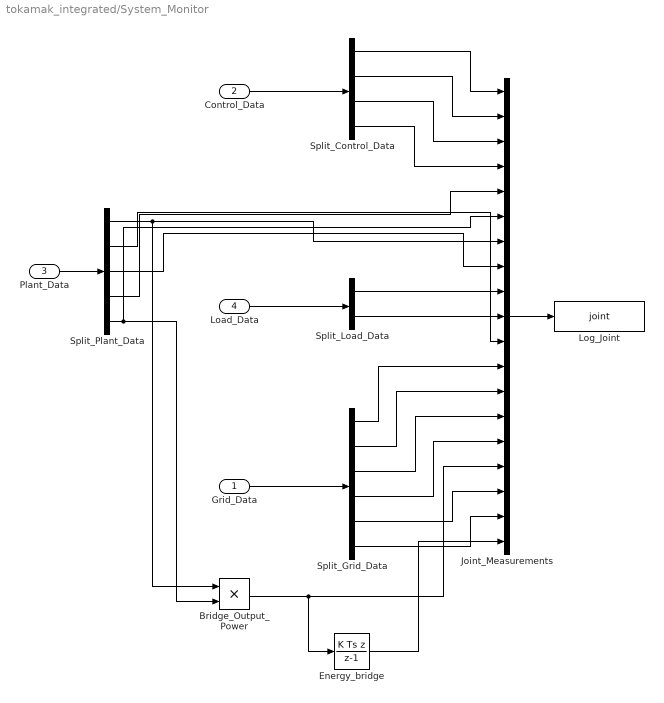
== system tokamak_integrated/System_Monitor ==
  Grid_Data : Inport
  Control_Data : Inport  Port=2
  Plant_Data : Inport  Port=3
  Load_Data : Inport  Port=4
  Bridge_Output_Power : Product
  Energy_bridge : DiscreteIntegrator  IntegratorMethod=Integration: Backward Euler  SampleTime=1e-6  ICPrevOutput=DiscIntNeverNeededParam  ICPrevScaledInput=DiscIntNeverNeededParam
  Joint_Measurements : Mux  Inputs=19
  Log_Joint : ToWorkspace  VariableName=joint  SaveFormat=Timeseries  SampleTime=1e-5
  Split_Control_Data : Demux
  Split_Grid_Data : Demux  Outputs=6
  Split_Load_Data : Demux  Outputs=2
  Split_Plant_Data : Demux  Outputs=5
  wires:
  Joint_Measurements/1 -> Log_Joint/1
  Energy_bridge/1 -> Joint_Measurements/19
  Bridge_Output_Power/1 -> Energy_bridge/1, Joint_Measurements/16
  Grid_Data/1 -> Split_Grid_Data/1
  Control_Data/1 -> Split_Control_Data/1
  Plant_Data/1 -> Split_Plant_Data/1
  Load_Data/1 -> Split_Load_Data/1
  Split_Control_Data/1 -> Joint_Measurements/1
  Split_Control_Data/2 -> Joint_Measurements/2
  Split_Control_Data/3 -> Joint_Measurements/3
  Split_Control_Data/4 -> Joint_Measurements/4
  Split_Plant_Data/4 -> Joint_Measurements/5
  Split_Plant_Data/5 -> Bridge_Output_Power/2, Joint_Measurements/6
  Split_Plant_Data/1 -> Bridge_Output_Power/1, Joint_Measurements/7
  Split_Plant_Data/3 -> Joint_Measurements/8
  Split_Load_Data/1 -> Joint_Measurements/9
  Split_Load_Data/2 -> Joint_Measurements/10
  Split_Plant_Data/2 -> Joint_Measurements/11
  Split_Grid_Data/1 -> Joint_Measurements/12
  Split_Grid_Data/2 -> Joint_Measurements/13
  Split_Grid_Data/3 -> Joint_Measurements/14
  Split_Grid_Data/4 -> Joint_Measurements/15
  Split_Grid_Data/5 -> Joint_Measurements/17
  Split_Grid_Data/6 -> Joint_Measurements/18

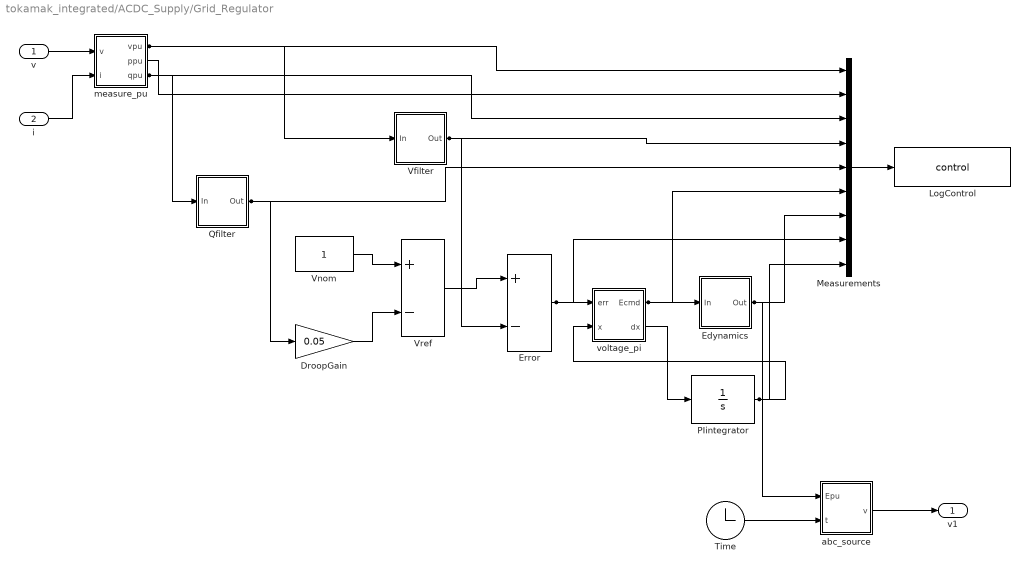
== system tokamak_integrated/ACDC_Supply/Grid_Regulator ==
  v : Inport
  i : Inport  Port=2
  DroopGain : Gain  Description=Implemented from the task-2 10 kV droop source guide.  Gain=0.05
  Edynamics : Subsystem  Description=Implemented from the task-2 10 kV droop source guide.
  Error : Sum  Description=Implemented from the task-2 10 kV droop source guide.  Inputs=+-
  LogControl : ToWorkspace  VariableName=control  SaveFormat=Timeseries  SampleTime=1e-4
      settings: Description=Implemented from the task-2 10 kV droop source guide.
  Measurements : Mux  Description=Implemented from the task-2 10 kV droop source guide.  Inputs=9
  PIintegrator : Integrator  Description=Guide initial condition is 0. Saturation hold test overrides to 0.15 via SimulationInput.
  Qfilter : Subsystem  Description=Implemented from the task-2 10 kV droop source guide.
  Time : Clock
      settings: Description=Implemented from the task-2 10 kV droop source guide.
  Vfilter : Subsystem  Description=Implemented from the task-2 10 kV droop source guide.
  Vnom : Constant  Description=Implemented from the task-2 10 kV droop source guide.
  Vref : Sum  Description=Implemented from the task-2 10 kV droop source guide.  Inputs=+-
  abc_source : MATLAB Function  Description=Implemented from the task-2 10 kV droop source guide.  TreatAsAtomicUnit=on
  measure_pu : MATLAB Function  Description=Implemented from the task-2 10 kV droop source guide.  TreatAsAtomicUnit=on
  voltage_pi : MATLAB Function  Description=Implemented from the task-2 10 kV droop source guide.  TreatAsAtomicUnit=on
  v1 : Outport
  wires:
  voltage_pi/1(Ecmd) -> Edynamics/1(In), Measurements/6
  Vref/1 -> Error/1
  Vnom/1 -> Vref/1
  Vfilter/1(Out) -> Error/2, Measurements/4
  PIintegrator/1 -> voltage_pi/2(x), Measurements/9
  Time/1 -> abc_source/2(t)
  v/1 -> measure_pu/1(v)
  measure_pu/3(qpu) -> Qfilter/1(In), Measurements/3
  Measurements/1 -> LogControl/1
  measure_pu/1(vpu) -> Vfilter/1(In), Measurements/1
  Qfilter/1(Out) -> Measurements/5, DroopGain/1
  Error/1 -> voltage_pi/1(err), Measurements/8
  voltage_pi/2(dx) -> PIintegrator/1
  Edynamics/1(Out) -> Measurements/7, abc_source/1(Epu)
  measure_pu/2(ppu) -> Measurements/2
  DroopGain/1 -> Vref/2
  abc_source/1(v) -> v1/1
  i/1 -> measure_pu/2(i)

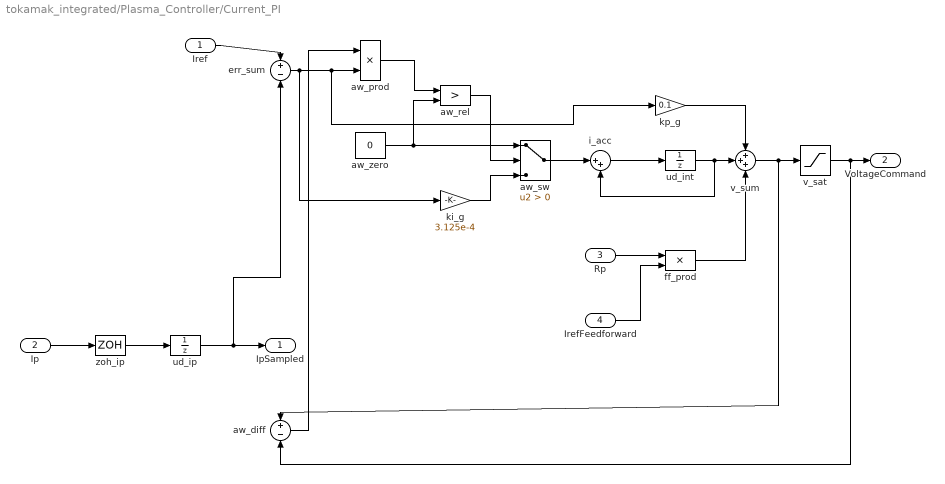
== system tokamak_integrated/Plasma_Controller/Current_PI ==
  Iref : Inport
  Ip : Inport  Port=2
  Rp : Inport  Port=3
  IrefFeedforward : Inport  Port=4
  aw_diff : Sum  Inputs=+-
  aw_prod : Product
  aw_rel : RelationalOperator  Operator=>  OutDataTypeStr=boolean  RndMeth=Simplest  InputSameDT=off
  aw_sw : Switch  Criteria=u2 > Threshold  SaturateOnIntegerOverflow=off  InputSameDT=off
  aw_zero : Constant  Value=0
  err_sum : Sum  Inputs=+-
  ff_prod : Product
  i_acc : Sum  Inputs=|++
  ki_g : Gain  Gain=3.125e-4
  kp_g : Gain  Gain=0.1
  ud_int : UnitDelay  SampleTime=50e-6
  ud_ip : UnitDelay  SampleTime=50e-6
  v_sat : Saturate  UpperLimit=400  LowerLimit=-400
  v_sum : Sum  Inputs=+++
  zoh_ip : ZeroOrderHold  SampleTime=50e-6
  IpSampled : Outport
  VoltageCommand : Outport  Port=2
  wires:
  ud_int/1 -> i_acc/2, v_sum/2
  ff_prod/1 -> v_sum/3
  err_sum/1 -> ki_g/1, aw_prod/2, kp_g/1
  kp_g/1 -> v_sum/1
  v_sum/1 -> v_sat/1, aw_diff/1
  IrefFeedforward/1 -> ff_prod/2
  Ip/1 -> zoh_ip/1
  Rp/1 -> ff_prod/1
  aw_sw/1 -> i_acc/1
  i_acc/1 -> ud_int/1
  ud_ip/1 -> IpSampled/1, err_sum/2
  v_sat/1 -> VoltageCommand/1, aw_diff/2
  ki_g/1 -> aw_sw/3
  Iref/1 -> err_sum/1
  aw_rel/1 -> aw_sw/2
  aw_zero/1 -> aw_rel/2, aw_sw/1
  aw_diff/1 -> aw_prod/1
  zoh_ip/1 -> ud_ip/1
  aw_prod/1 -> aw_rel/1

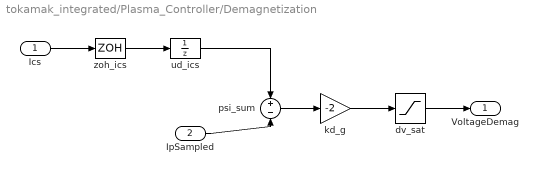
== system tokamak_integrated/Plasma_Controller/Demagnetization ==
  Ics : Inport
  IpSampled : Inport  Port=2
  dv_sat : Saturate  UpperLimit=400  LowerLimit=-400
  kd_g : Gain  Gain=-2
  psi_sum : Sum  Inputs=+-
  ud_ics : UnitDelay  SampleTime=50e-6
  zoh_ics : ZeroOrderHold  SampleTime=50e-6
  VoltageDemag : Outport
  wires:
  dv_sat/1 -> VoltageDemag/1
  ud_ics/1 -> psi_sum/1
  zoh_ics/1 -> ud_ics/1
  Ics/1 -> zoh_ics/1
  IpSampled/1 -> psi_sum/2
  kd_g/1 -> dv_sat/1
  psi_sum/1 -> kd_g/1

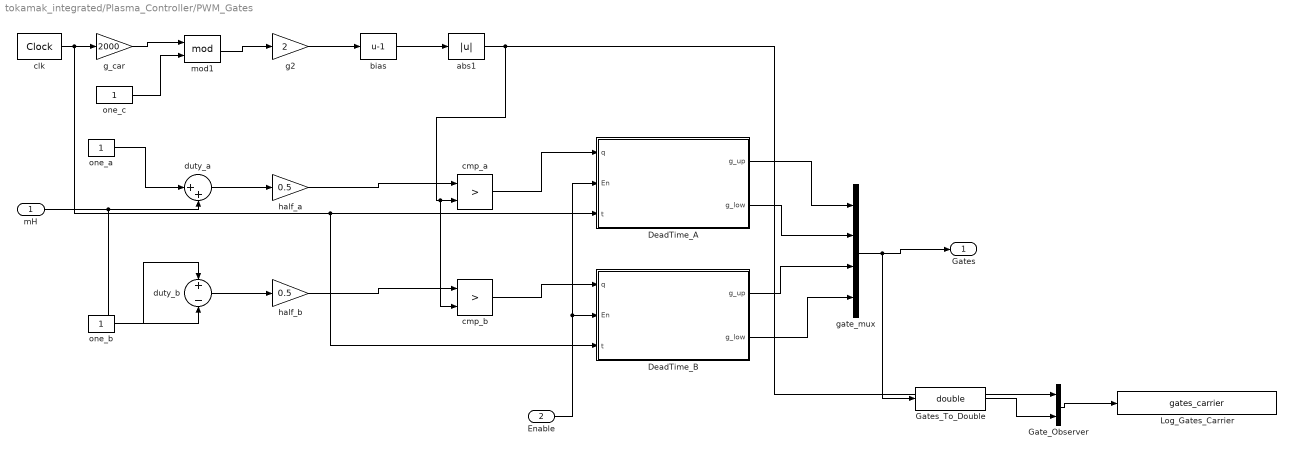
== system tokamak_integrated/Plasma_Controller/PWM_Gates ==
  mH : Inport
  Enable : Inport  Port=2
  DeadTime_A : Subsystem
  DeadTime_B : Subsystem
  Gate_Observer : Mux  Inputs=2
  Gates_To_Double : DataTypeConversion  OutDataTypeStr=double  SaturateOnIntegerOverflow=off  RndMeth=Floor
  Log_Gates_Carrier : ToWorkspace  VariableName=gates_carrier  SaveFormat=Timeseries  SampleTime=-1
      settings: MaxDataPoints=20001
  abs1 : Abs  SaturateOnIntegerOverflow=off
  bias : Bias  Bias=-1  SaturateOnIntegerOverflow=off
  clk : DigitalClock  SampleTime=1e-6
  cmp_a : RelationalOperator  Operator=>  OutDataTypeStr=boolean  RndMeth=Simplest  InputSameDT=off
  cmp_b : RelationalOperator  Operator=>  OutDataTypeStr=boolean  RndMeth=Simplest  InputSameDT=off
  duty_a : Sum  Inputs=|++
  duty_b : Sum  Inputs=+-
  g2 : Gain  Gain=2
  g_car : Gain  Gain=2000
  gate_mux : Mux
  half_a : Gain  Gain=0.5
  half_b : Gain  Gain=0.5
  mod1 : Math  Operator=mod
  one_a : Constant
  one_b : Constant
  one_c : Constant
  Gates : Outport
  wires:
  DeadTime_A/1(g_up) -> gate_mux/1
  Enable/1 -> DeadTime_B/2(En), DeadTime_A/2(En)
  cmp_b/1 -> DeadTime_B/1(q)
  cmp_a/1 -> DeadTime_A/1(q)
  clk/1 -> g_car/1, DeadTime_A/3(t), DeadTime_B/3(t)
  gate_mux/1 -> Gates/1, Gates_To_Double/1
  DeadTime_A/2(g_low) -> gate_mux/2
  DeadTime_B/1(g_up) -> gate_mux/3
  DeadTime_B/2(g_low) -> gate_mux/4
  Gate_Observer/1 -> Log_Gates_Carrier/1
  abs1/1 -> Gate_Observer/1, cmp_b/2, cmp_a/2
  Gates_To_Double/1 -> Gate_Observer/2
  bias/1 -> abs1/1
  half_a/1 -> cmp_a/1
  half_b/1 -> cmp_b/1
  mH/1 -> duty_b/2, duty_a/2
  duty_a/1 -> half_a/1
  g2/1 -> bias/1
  one_c/1 -> mod1/2
  duty_b/1 -> half_b/1
  one_a/1 -> duty_a/1
  g_car/1 -> mod1/1
  one_b/1 -> duty_b/1
  mod1/1 -> g2/1

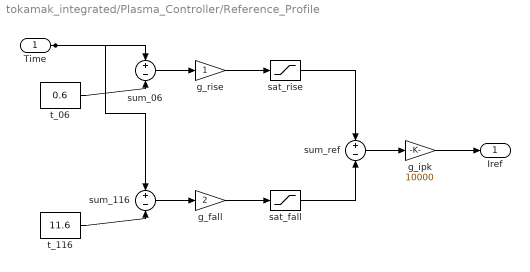
== system tokamak_integrated/Plasma_Controller/Reference_Profile ==
  Time : Inport
  g_fall : Gain  Gain=2
  g_ipk : Gain  Gain=10000
  g_rise : Gain
  sat_fall : Saturate  UpperLimit=1  LowerLimit=0
  sat_rise : Saturate  UpperLimit=1  LowerLimit=0
  sum_06 : Sum  Inputs=+-
  sum_116 : Sum  Inputs=+-
  sum_ref : Sum  Inputs=+-
  t_06 : Constant  Value=0.6
  t_116 : Constant  Value=11.6
  Iref : Outport
  wires:
  sum_116/1 -> g_fall/1
  t_116/1 -> sum_116/2
  sum_ref/1 -> g_ipk/1
  t_06/1 -> sum_06/2
  Time/1 -> sum_116/1, sum_06/1
  sat_fall/1 -> sum_ref/2
  sat_rise/1 -> sum_ref/1
  g_ipk/1 -> Iref/1
  sum_06/1 -> g_rise/1
  g_rise/1 -> sat_rise/1
  g_fall/1 -> sat_fall/1

== system tokamak_integrated/ACDC_Supply/Grid_Regulator/Edynamics ==
  In : Inport
  Difference : Sum  Inputs=+-
  Rate : Gain  Gain=20
  State : Integrator  InitialCondition=1
  Out : Outport
  wires:
  In/1 -> Difference/1
  Difference/1 -> Rate/1
  Rate/1 -> State/1
  State/1 -> Out/1, Difference/2

== system tokamak_integrated/ACDC_Supply/Grid_Regulator/Qfilter ==
  In : Inport
  Difference : Sum  Inputs=+-
  Rate : Gain  Gain=50
  State : Integrator
  Out : Outport
  wires:
  In/1 -> Difference/1
  Difference/1 -> Rate/1
  Rate/1 -> State/1
  State/1 -> Out/1, Difference/2

== system tokamak_integrated/ACDC_Supply/Grid_Regulator/Vfilter ==
  In : Inport
  Difference : Sum  Inputs=+-
  Rate : Gain  Gain=100
  State : Integrator  InitialCondition=1
  Out : Outport
  wires:
  In/1 -> Difference/1
  Difference/1 -> Rate/1
  Rate/1 -> State/1
  State/1 -> Out/1, Difference/2

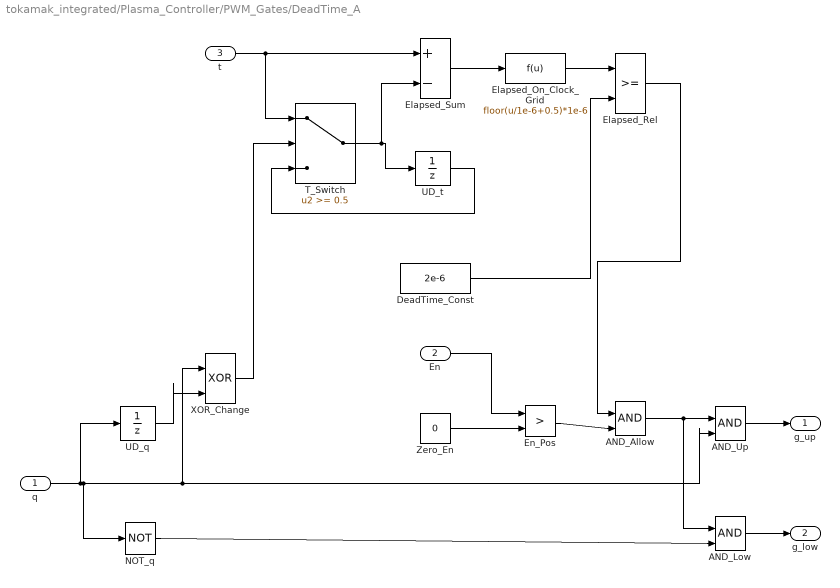
== system tokamak_integrated/Plasma_Controller/PWM_Gates/DeadTime_A ==
  q : Inport
  En : Inport  Port=2
  t : Inport  Port=3
  AND_Allow : Logic  IconShape=distinctive  AllPortsSameDT=off  OutDataTypeStr=boolean
  AND_Low : Logic  IconShape=distinctive  AllPortsSameDT=off  OutDataTypeStr=boolean
  AND_Up : Logic  IconShape=distinctive  AllPortsSameDT=off  OutDataTypeStr=boolean
  DeadTime_Const : Constant  Value=2e-6
  Elapsed_On_Clock_Grid : Fcn  Expr=floor(u/1e-6+0.5)*1e-6
  Elapsed_Rel : RelationalOperator  OutDataTypeStr=boolean  RndMeth=Simplest  InputSameDT=off
  Elapsed_Sum : Sum  Inputs=+-
  En_Pos : RelationalOperator  Operator=>  OutDataTypeStr=boolean  RndMeth=Simplest  InputSameDT=off
  NOT_q : Logic  Operator=NOT  Inputs=1  IconShape=distinctive  AllPortsSameDT=off  OutDataTypeStr=boolean
  T_Switch : Switch  Threshold=0.5  SaturateOnIntegerOverflow=off  InputSameDT=off
  UD_q : UnitDelay  SampleTime=1e-6
  UD_t : UnitDelay  InitialCondition=-1  SampleTime=1e-6
  XOR_Change : Logic  Operator=XOR  IconShape=distinctive  AllPortsSameDT=off  OutDataTypeStr=boolean
  Zero_En : Constant  Value=0
  g_up : Outport
  g_low : Outport  Port=2
  wires:
  AND_Low/1 -> g_low/1
  AND_Up/1 -> g_up/1
  NOT_q/1 -> AND_Low/2
  AND_Allow/1 -> AND_Up/1, AND_Low/1
  En_Pos/1 -> AND_Allow/2
  Zero_En/1 -> En_Pos/2
  En/1 -> En_Pos/1
  T_Switch/1 -> UD_t/1, Elapsed_Sum/2
  UD_t/1 -> T_Switch/3
  XOR_Change/1 -> T_Switch/2
  t/1 -> Elapsed_Sum/1, T_Switch/1
  UD_q/1 -> XOR_Change/2
  q/1 -> AND_Up/2, XOR_Change/1, NOT_q/1, UD_q/1
  Elapsed_On_Clock_Grid/1 -> Elapsed_Rel/1
  Elapsed_Sum/1 -> Elapsed_On_Clock_Grid/1
  DeadTime_Const/1 -> Elapsed_Rel/2
  Elapsed_Rel/1 -> AND_Allow/1

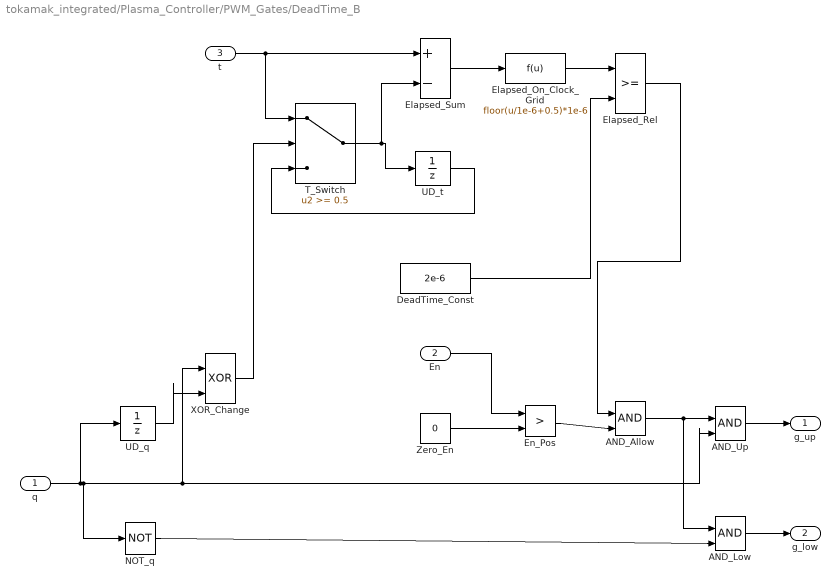
== system tokamak_integrated/Plasma_Controller/PWM_Gates/DeadTime_B ==
  q : Inport
  En : Inport  Port=2
  t : Inport  Port=3
  AND_Allow : Logic  IconShape=distinctive  AllPortsSameDT=off  OutDataTypeStr=boolean
  AND_Low : Logic  IconShape=distinctive  AllPortsSameDT=off  OutDataTypeStr=boolean
  AND_Up : Logic  IconShape=distinctive  AllPortsSameDT=off  OutDataTypeStr=boolean
  DeadTime_Const : Constant  Value=2e-6
  Elapsed_On_Clock_Grid : Fcn  Expr=floor(u/1e-6+0.5)*1e-6
  Elapsed_Rel : RelationalOperator  OutDataTypeStr=boolean  RndMeth=Simplest  InputSameDT=off
  Elapsed_Sum : Sum  Inputs=+-
  En_Pos : RelationalOperator  Operator=>  OutDataTypeStr=boolean  RndMeth=Simplest  InputSameDT=off
  NOT_q : Logic  Operator=NOT  Inputs=1  IconShape=distinctive  AllPortsSameDT=off  OutDataTypeStr=boolean
  T_Switch : Switch  Threshold=0.5  SaturateOnIntegerOverflow=off  InputSameDT=off
  UD_q : UnitDelay  SampleTime=1e-6
  UD_t : UnitDelay  InitialCondition=-1  SampleTime=1e-6
  XOR_Change : Logic  Operator=XOR  IconShape=distinctive  AllPortsSameDT=off  OutDataTypeStr=boolean
  Zero_En : Constant  Value=0
  g_up : Outport
  g_low : Outport  Port=2
  wires:
  AND_Low/1 -> g_low/1
  AND_Up/1 -> g_up/1
  NOT_q/1 -> AND_Low/2
  AND_Allow/1 -> AND_Up/1, AND_Low/1
  En_Pos/1 -> AND_Allow/2
  Zero_En/1 -> En_Pos/2
  En/1 -> En_Pos/1
  T_Switch/1 -> UD_t/1, Elapsed_Sum/2
  UD_t/1 -> T_Switch/3
  XOR_Change/1 -> T_Switch/2
  t/1 -> Elapsed_Sum/1, T_Switch/1
  UD_q/1 -> XOR_Change/2
  q/1 -> AND_Up/2, XOR_Change/1, NOT_q/1, UD_q/1
  Elapsed_On_Clock_Grid/1 -> Elapsed_Rel/1
  Elapsed_Sum/1 -> Elapsed_On_Clock_Grid/1
  DeadTime_Const/1 -> Elapsed_Rel/2
  Elapsed_Rel/1 -> AND_Allow/1

== matlab function tokamak_integrated/ACDC_Supply/Grid_Regulator/abc_source ==
  data: Epu input; v output; t input
function v = abc_source(Epu,t)
Vll=10000*Epu;
th=2*pi*50*t;
v=sqrt(2/3)*Vll*[sin(th);sin(th-2*pi/3);sin(th+2*pi/3)];
end

== matlab function tokamak_integrated/ACDC_Supply/Grid_Regulator/measure_pu ==
  data: v input; vpu output; i input; ppu output; qpu output
function [vpu,ppu,qpu] = measure_pu(v,i)
va=(2/3)*(v(1)-0.5*v(2)-0.5*v(3));
vb=(2/3)*(sqrt(3)/2)*(v(2)-v(3));
ia=(2/3)*(i(1)-0.5*i(2)-0.5*i(3));
ib=(2/3)*(sqrt(3)/2)*(i(2)-i(3));
vpu=sqrt(1.5*(va*va+vb*vb))/10000;
ppu=(v(1)*i(1)+v(2)*i(2)+v(3)*i(3))/1e7;
qpu=1.5*(vb*ia-va*ib)/1e7;
end

== matlab function tokamak_integrated/ACDC_Supply/Grid_Regulator/voltage_pi ==
  data: err input; Ecmd output; x input; dx output
function [Ecmd,dx] = voltage_pi(err,x)
raw=0.5*err+x;
u=min(max(raw,-0.15),0.15);
dx=10*err;
if (raw>=0.15 && err>0)||(raw<=-0.15 && err<0)
 dx=0;
end
Ecmd=1+u;
end
